simulink model "model_Lab3"  (R2024a)
settings: Solver=VariableStepAuto  StartTime=0.0  StopTime=90  RelTol=1e-3
values from neighbouring files (symbols this model uses):
  k1 = -1.9731    [evaluate_controller.m]
  k2 = 0.0609    [evaluate_controller.m]    (also in system_ID_Lab2.m)
  k3 = -4.838    [evaluate_controller.m]
  m0i = f0i*T - f1i    [evaluate_controller.m]
  m0o = -f3o + f2o*T - f1o*T^2 + f0o*T^3    [evaluate_controller.m]
  m1i = f1i    (= 1)    [evaluate_controller.m]
  m1o = 3*f3o - 2*f2o*T + f1o*T^2    [evaluate_controller.m]
  m2o = -3*f3o + f2o*T    [evaluate_controller.m]
  m3o = f3o    (= 1)    [evaluate_controller.m]
  n0i = g0i*T - g1i    [evaluate_controller.m]
  n0o = -g3o + g2o*T - g1o*T^2 + g0o*T^3    [evaluate_controller.m]
  n1i = g1i    [evaluate_controller.m]
  n1o = 3*g3o - 2*g2o*T + g1o*T^2    [evaluate_controller.m]
  n2o = -3*g3o + g2o*T    [evaluate_controller.m]
  n3o = g3o    (= 0)    [evaluate_controller.m]
  T = 0.001    [evaluate_controller.m]
  tau = 0.02387    [evaluate_controller.m]    (also in system_ID_Lab1.m = 1 / (2 * zeta * wn))
settings Model: Creator=michael  LastModifiedBy=michael

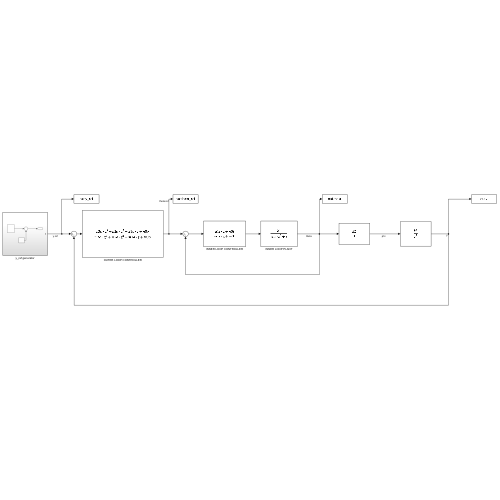
[thumbnail: Simulink's stored preview of the top-level diagram]
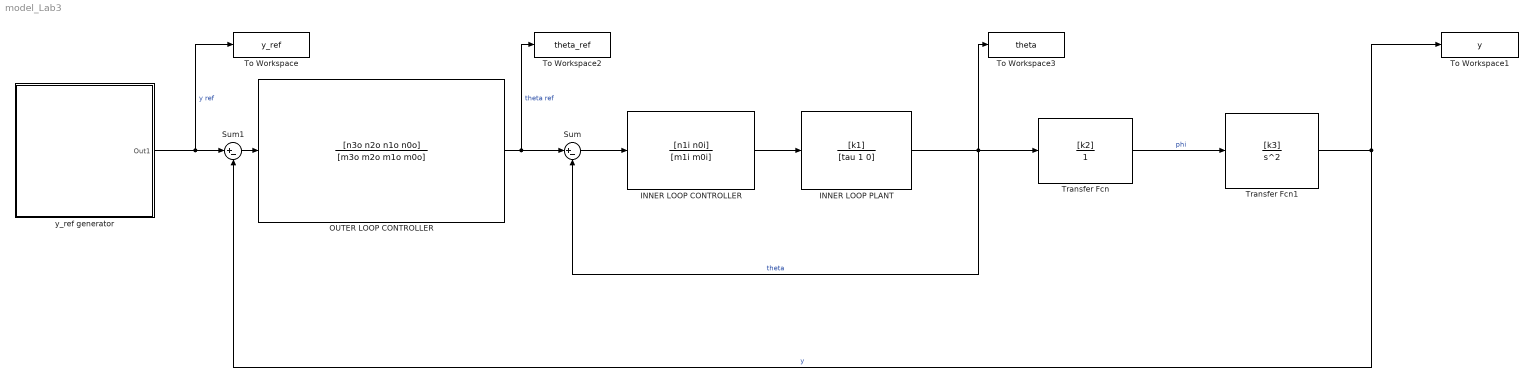
== system model_Lab3 ==
  INNER LOOP CONTROLLER : DiscreteTransferFcn  Numerator=[n1i n0i]  Denominator=[m1i m0i]  SampleTime=T
  INNER LOOP PLANT : TransferFcn  Numerator=[k1]  Denominator=[tau 1 0]
  OUTER LOOP CONTROLLER : DiscreteTransferFcn  Numerator=[n3o n2o n1o n0o]  Denominator=[m3o m2o m1o m0o]  SampleTime=T
  Sum : Sum  Inputs=|+-
  Sum1 : Sum  Inputs=|+-
  To Workspace : ToWorkspace  VariableName=y_ref  SaveFormat=Timeseries  SampleTime=-1
  To Workspace1 : ToWorkspace  VariableName=y  SaveFormat=Timeseries  SampleTime=-1
  To Workspace2 : ToWorkspace  VariableName=theta_ref  SaveFormat=Timeseries  SampleTime=-1
  To Workspace3 : ToWorkspace  VariableName=theta  SaveFormat=Timeseries  SampleTime=-1
  Transfer Fcn : TransferFcn  Numerator=[k2]  Denominator=[1]
  Transfer Fcn1 : TransferFcn  Numerator=[k3]  Denominator=[1 0 0]
  y_ref generator : Subsystem
  wires:
  INNER LOOP PLANT/1 -> Sum/2, To Workspace3/1, Transfer Fcn/1  "theta"
  INNER LOOP CONTROLLER/1 -> INNER LOOP PLANT/1
  OUTER LOOP CONTROLLER/1 -> Sum/1, To Workspace2/1  "theta ref"
  Sum/1 -> INNER LOOP CONTROLLER/1
  Transfer Fcn/1 -> Transfer Fcn1/1  "phi"
  y_ref generator/1(Out1) -> To Workspace/1, Sum1/1  "y ref"
  Sum1/1 -> OUTER LOOP CONTROLLER/1
  Transfer Fcn1/1 -> Sum1/2, To Workspace1/1  "y"

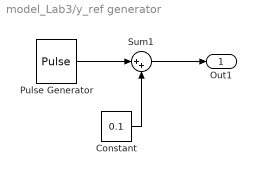
== system model_Lab3/y_ref generator ==
  Constant : Constant  Value=0.1
  Pulse Generator : DiscretePulseGenerator  PulseType=Time based  Amplitude=0.15  Period=30  PulseWidth=50
  Sum1 : Sum  Inputs=|++
  Out1 : Outport
  wires:
  Constant/1 -> Sum1/2
  Pulse Generator/1 -> Sum1/1
  Sum1/1 -> Out1/1
